simulink model "Communication_rate_control"  (R2025a)
settings: Solver=VariableStepAuto  StartTime=0.0  StopTime=30  RelTol=1e-3
InitFcn:
  | %% Simulation parameters and waypoint trajectory
  | % Initial drone positions.
  | init_0=[0;0;0];
  | d_s=4;
  | init_1=init_0+d_s*[-1;0.1;0];
  | init_2=init_0+d_s*[0.3;-2;0];
  | init_3=init_0+d_s*[0.2;3;0];
  | init_4=init_0+d_s*[4;0.4;0];
  | 
  | Threshold = 1000*ones(45,1);
  | for i=1:9:37
  |     Threshold(i:i+2)=10;
  | end
  | gain_2=1;
  | 
  | % PID controller gains.
  | PID_p=20;
  | PID_i=50;
  | PID_d=0;
  | 
  | % Router queues and background traffic.
  | router_buffer=50;
  | router_bandwith=25;
  | router_init_queue=[2,0,0,0,0];
  | traffic_mean=20;
  | traffic_variance=1;
  | 
  | 
  | % Desired formation offsets.
  | init_f_0=[0;0;0];
  | d_f=1;
  | init_f_1=init_0+d_f*[-1;0;0];
  | init_f_2=init_0+d_f*[0;-1;0];
  | init_f_3=init_0+d_f*[0;1;0];
  | init_f_4=init_0+d_f*[1;0;0];
  | 
  | % Quadrotor mass and inertia.
  | mass = 1.2;
  | Ib   = diag([1.2416 1.2416 2*1.2416]);
  | 
  | % Time grid and waypoint trajectory.
  | Ts        = 0.001;
  | ttot      = 20;
  | tdead     = 10;
  | totalTime = ttot + tdead;
  | Nsamples  = 3000;
  | t_sample  = linspace(0, totalTime, Nsamples);
  | t=t_sample;
  | waypoints = [ ...
  |              0  0 -2 0;
  |              3  4 -5 0;
  |              2  1 -8 0;
  |              0 0 -20 0];
  | 
  | M    = size(waypoints,1);
  | t_wp = linspace(0, ttot, M);
  | 
  | p_d      = zeros(4, Nsamples);
  | dot_p_d  = zeros(4, Nsamples);
  | ddot_p_d = zeros(4, Nsamples);
  | ... (+33 lines)
undefined symbols (not defined in the file): A_diacenza, DiscIntNeverNeededParam, K, L
libraries: dspsigops x10, robotcorelib x5, slpidlib x5, dspstat3 x5, uavutilslib x1
(part 2 of 3)

== system Communication_rate_control/Subsystem1/Subsystem_5 ==
  References : Inport
  Coordinate Transformation Conversion : robotcorelib/Coordinate Transformation Conversion  InputRepresentation=Rotation Matrix  InputEulerSequence=ZYX  ShowTrVecInputPort=on  OutputRepresentation=Quaternion  OutputEulerSequence=ZYX  ShowTrVecOutputPort=on  SimulateUsing=Interpreted execution
  Inner-loop control : Subsystem
  Outer-loop control : MATLAB Function  TreatAsAtomicUnit=on
  Planner : Subsystem
  Quadrotor dynamics : Subsystem
  Scope{,1..5} (6 alike) : Scope
      Scope settings: ActiveDisplayYMinimum=-1.2E-5  ActiveDisplayYMaximum=1.2E-5
      Scope1 settings: ActiveDisplayYMinimum=-1.2E-5  ActiveDisplayYMaximum=1.2E-5
      Scope2 settings: ActiveDisplayYMinimum=-3.9E-5  ActiveDisplayYMaximum=1.1E-5  DataLoggingVariableName=ScopeData2
      Scope3 settings: ActiveDisplayYMinimum=-0.00022  ActiveDisplayYMaximum=0.00011  DataLoggingVariableName=ScopeData3
      Scope4 settings: ActiveDisplayYMinimum=11.66748  ActiveDisplayYMaximum=12.03695  DataLoggingVariableName=ScopeData4
      Scope5 settings: ActiveDisplayYMinimum=-0.02035  ActiveDisplayYMaximum=0.02036  DataLoggingVariableName=ScopeData5
  Terminator : Terminator
  Terminator3 : Terminator
  Unit Delay1 u0=12N : UnitDelay  InitialCondition=12  SampleTime=Ts
  Unit Delay2 : UnitDelay  InitialCondition=[0 0 0]  SampleTime=Ts
  Zero-Order Hold{1..5} (5 alike) : ZeroOrderHold  SampleTime=Ts
  Lin Acc : Outport
  Lin Vel : Outport  Port=2
  Lin Pos : Outport  Port=3
  Rotation : Outport  Port=4
  wires:
  Zero-Order Hold5/1 -> Lin Acc/1
  Quadrotor dynamics/7(lin_acc) -> Zero-Order Hold5/1
  Planner/1(position_des) -> Outer-loop control/4(position_des)
  Quadrotor dynamics/1(Position) -> Zero-Order Hold4/1
  Quadrotor dynamics/3(Rb) -> Zero-Order Hold2/1, Coordinate Transformation Conversion/1
  Quadrotor dynamics/4(dot_Rb) -> Terminator/1
  Planner/4(xb_des) -> Inner-loop control/4(xb_des)
  Inner-loop control/1(tau) -> Unit Delay2/1
  Planner/2(linear_velocity_des) -> Outer-loop control/5(vel_linear_des)
  Quadrotor dynamics/2(Linear_velocity) -> Zero-Order Hold1/1
  Quadrotor dynamics/6(dot_omega_bb) -> Terminator3/1
  Outer-loop control/3(err_p) -> Scope2/1
  Coordinate Transformation Conversion/1 -> Rotation/1
  Quadrotor dynamics/5(omega_bb) -> Zero-Order Hold3/1
  Zero-Order Hold2/1 -> Inner-loop control/2(Rb), Outer-loop control/3(Rb)
  References/1 -> Planner/1(References)
  Planner/3(linear_acceleration_des) -> Outer-loop control/6(acc_linear_des)
  Inner-loop control/3(err_W) -> Scope1/1
  Outer-loop control/2(zb_des) -> Inner-loop control/1(zb_des)
  Inner-loop control/2(err_R) -> Scope/1
  Outer-loop control/1(uT) -> Unit Delay1 u0=12N/1
  Unit Delay2/1 -> Quadrotor dynamics/2(tau_b), Scope5/1
  Zero-Order Hold3/1 -> Inner-loop control/3(omega_bb)
  Unit Delay1 u0=12N/1 -> Scope4/1, Quadrotor dynamics/1(uT)
  Outer-loop control/4(dot_err_p) -> Scope3/1
  Zero-Order Hold1/1 -> Outer-loop control/2(linear_vel), Lin Vel/1
  Zero-Order Hold4/1 -> Outer-loop control/1(position), Lin Pos/1

== system Communication_rate_control/Subsystem13/Planner ==
  Constant : Constant  Value=0
  Mux{1..4} (4 alike) : Mux  Inputs=3
  Trigonometric Function : Trigonometry
  Trigonometric Function1 : Trigonometry  Operator=cos
  ddot_x_d : FromWorkspace  VariableName=[t' ddot_csi_d(1,:)']  SampleTime=Ts
  ddot_y_d : FromWorkspace  VariableName=[t' ddot_csi_d(2,:)']  SampleTime=Ts
  ddot_z_d : FromWorkspace  VariableName=[t' ddot_csi_d(3,:)']  SampleTime=Ts
  dot_x_d1 : FromWorkspace  VariableName=[t' dot_csi_d(1,:)']  SampleTime=Ts
  dot_y_d1 : FromWorkspace  VariableName=[t' dot_csi_d(2,:)']  SampleTime=Ts
  dot_z_d1 : FromWorkspace  VariableName=[t' dot_csi_d(3,:)']  SampleTime=Ts
  psi_d1 : FromWorkspace  VariableName=[t' psi_d']  SampleTime=Ts
  x_d : FromWorkspace  VariableName=[t' csi_d(1,:)']  SampleTime=Ts
  y_d : FromWorkspace  VariableName=[t' csi_d(2,:)']  SampleTime=Ts
  z_d : FromWorkspace  VariableName=[t' csi_d(3,:)']  SampleTime=Ts
  position_des : Outport
  linear_velocity_des : Outport  Port=2
  linear_acceleration_des : Outport  Port=3
  xb_des : Outport  Port=4
  wires:
  y_d/1 -> Mux1/2
  z_d/1 -> Mux1/3
  x_d/1 -> Mux1/1
  ddot_y_d/1 -> Mux2/2
  ddot_z_d/1 -> Mux2/3
  ddot_x_d/1 -> Mux2/1
  Mux2/1 -> linear_acceleration_des/1
  Mux1/1 -> position_des/1
  dot_y_d1/1 -> Mux3/2
  dot_z_d1/1 -> Mux3/3
  dot_x_d1/1 -> Mux3/1
  Mux3/1 -> linear_velocity_des/1
  Mux4/1 -> xb_des/1
  Trigonometric Function/1 -> Mux4/2
  psi_d1/1 -> Trigonometric Function/1, Trigonometric Function1/1
  Trigonometric Function1/1 -> Mux4/1
  Constant/1 -> Mux4/3

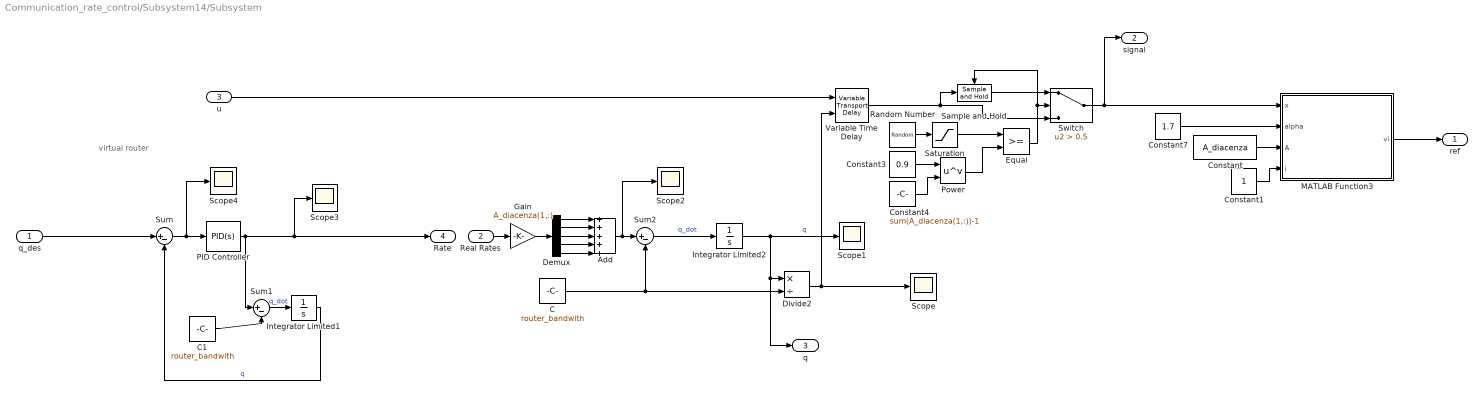
== system Communication_rate_control/Subsystem14/Subsystem ==
  note: virtual router
  q_des : Inport
  " Real Rates" : Inport  Port=2
  u : Inport  Port=3
  Add : Sum  Inputs=+++++
  C : Constant  Value=router_bandwith
  C1 : Constant  Value=router_bandwith
  Constant : Constant  Value=A_diacenza
  Constant1 : Constant
  Constant3 : Constant  Value=0.9
  Constant4 : Constant  Value=sum(A_diacenza(1,:))-1
  Constant7 : Constant  Value=1.7
  Demux : Demux  Outputs=5
  Divide2 : Product  Inputs=*/
  Equal : RelationalOperator  OutDataTypeStr=boolean  RndMeth=Simplest  InputSameDT=off
  Gain : Gain  Gain=A_diacenza(1,:)
  Integrator Limited1 : Integrator  InitialCondition=router_init_queue(1)  LimitOutput=on  UpperSaturationLimit=router_buffer  LowerSaturationLimit=0
  Integrator Limited2 : Integrator  InitialCondition=router_init_queue(1)  LimitOutput=on  UpperSaturationLimit=router_buffer  LowerSaturationLimit=0
  MATLAB Function3 : MATLAB Function  TreatAsAtomicUnit=on
  PID Controller : slpidlib/PID Controller  Controller=PID  Form=Parallel  TimeDomain=Continuous-time  UseExternalTs=off  SampleTime=-1  IntegratorMethod=Forward Euler  FilterMethod=Forward Euler  ControllerParametersSource=internal  P=PID_p  I=PID_i  UseKiTs=off  D=PID_d  UseExternalDerivativeSource=off  N=100  UseFilter=on  TunerSelectOption=Transfer Function Based (PID Tuner App)  InitialConditionSource=internal  InitialConditionForIntegrator=0  InitialConditionForFilter=0  DifferentiatorICPrevScaledInput=0  ExternalReset=none  TrackingMode=off  Kt=1  LimitOutput=off  SatLimitsSource=internal  UpperSaturationLimit=inf  LowerSaturationLimit=-inf  LinearizeAsGain=on  AntiWindupMode=none  Kb=1  LimitIntegrator=off  UpperIntegratorSaturationLimit=inf  LowerIntegratorSaturationLimit=-inf  POutMin=[]  POutMax=[]  IOutMin=[]  IOutMax=[]  DOutMin=[]  DOutMax=[]  NOutMin=[]  NOutMax=[]  SumOutMin=[]  SumOutMax=[]  SaturationOutMin=[]  SaturationOutMax=[]  PParamMin=[]  PParamMax=[]  IParamMin=[]  IParamMax=[]  DParamMin=[]  DParamMax=[]  NParamMin=[]  NParamMax=[]  KbParamMin=[]  KbParamMax=[]  KtParamMin=[]  KtParamMax=[]  KbOutMin=[]  KbOutMax=[]  KtOutMin=[]  KtOutMax=[]  IntegratorOutMin=[]  IntegratorOutMax=[]  FilterOutMin=[]  FilterOutMax=[]  SumI1OutMin=[]  SumI1OutMax=[]  SumI2OutMin=[]  SumI2OutMax=[]  SumI3OutMin=[]  SumI3OutMax=[]  SumI4OutMin=[]  SumI4OutMax=[]  SumDOutMin=[]  SumDOutMax=[]  DifferentiatorOutMin=[]  DifferentiatorOutMax=[]  FilterDiffOutCoefMin=[]  FilterDiffOutCoefMax=[]  ReciprocalOutMin=[]  ReciprocalOutMax=[]  SumDenOutMin=[]  SumDenOutMax=[]  SumNumOutMin=[]  SumNumOutMax=[]  DivideOutMin=[]  DivideOutMax=[]  UdiffTsProdOutMin=[]  UdiffTsProdOutMax=[]  NTsProdOutMin=[]  NTsProdOutMax=[]  UintegralTsProdOutMin=[]  UintegralTsProdOutMax=[]  UngainTsProdOutMin=[]  UngainTsProdOutMax=[]  ClampingZeroOutDataTypeStr=Inherit: Inherit via back propagation  ClampingZeroOutMin=[]  ClampingZeroOutMax=[]  FilterDenConstantOutDataTypeStr=Inherit: Inherit via back propagation  FilterDenConstantOutMin=[]  FilterDenConstantOutMax=[]  PCopyOutDataTypeStr=Inherit: Inherit via back propagation  PCopyOutMin=[]  PCopyOutMax=[]  NCopyOutDataTypeStr=Inherit: Inherit via back propagation  NCopyOutMin=[]  NCopyOutMax=[]  IntegratorContinuousStateAttributes=''  IntegratorStateMustResolveToSignalObject=off  IntegratorRTWStateStorageClass=Auto  FilterContinuousStateAttributes=''  FilterStateMustResolveToSignalObject=off  FilterRTWStateStorageClass=Auto  ParallelPVariant=InternalParameters  IdealPVariant=Disabled  IVariant=InternalParameters  DVariant=InternalParameters  IntegratorVariant=Continuous  SatVariant=Disabled  AWVariant=Passthrough  PCopyVariant=Disabled  TRVariant=Disabled  FdbkBlocksVariant=Forward  IdealPFdbkVariant=Disabled  SatFdbkVariant=Disabled  DerivativeFilterVariant=ContFilter  NVariant=InternalParameters  NCopyVariant=Disabled  FilterICVariant=InternalICsFilter  IntegratorICVariant=InternalICs  ExternalResetVariant=Disabled  TRSumVariant=Passthrough  SumFdbkVariant=Disabled  SumVariant=Sum_PID  TsampFilterVariant=InternalTs  TsampNgainVariant=Passthrough  TsampIntegralVariant=Disabled_SignalSpec  ExternalSaturationOutDataTypeStr=Inherit: Same as second input  DerivativeSourceVariant=ErrorSignal  PreIntVariant=InternalPreInt
  Power : Math  Operator=pow
  Random Number : RandomNumber  Mean=0.5  Variance=0.5  SampleTime=0.1
  Sample and Hold : dspsigops/Sample and Hold  trig=Rising edge  initCond=0  latchinput=off
  Saturation : Saturate  UpperLimit=1  LowerLimit=0
  Scope{,1..4} (5 alike) : Scope
      Scope settings: ActiveDisplayYMinimum=-1  ActiveDisplayYMaximum=1  DataLoggingVariableName=ScopeData7
      Scope1 settings: ActiveDisplayYMinimum=-1  ActiveDisplayYMaximum=1  DataLoggingVariableName=ScopeData8
      Scope2 settings: ActiveDisplayYMinimum=13.95346208966077  ActiveDisplayYMaximum=109.54638870962908  DataLoggingVariableName=ScopeData13
      Scope3 settings: ActiveDisplayYMinimum=18.031914924971169  ActiveDisplayYMaximum=21.223404282118214  DataLoggingVariableName=ScopeData12
      Scope4 settings: ActiveDisplayYMinimum=-3.625  ActiveDisplayYMaximum=2.625  DataLoggingVariableName=ScopeData29
  Sum : Sum  Inputs=|+-
  Sum1 : Sum  Inputs=|+-
  Sum2 : Sum  Inputs=|+-
  Switch : Switch  Criteria=u2 > Threshold  Threshold=0.5  SaturateOnIntegerOverflow=off  InputSameDT=off
  Variable Time Delay : VariableTransportDelay  MaximumDelay=1000  InitialOutput=[init_0;zeros(6,1);init_1;zeros(6,1);init_2;zeros(6,1);init_3;zeros(6,1);init_4;zeros(6,1);]  MaximumPoints=1e4  ZeroDelay=on
  ref : Outport
  "signal " : Outport  Port=2
  q : Outport  Port=3
  " Rate" : Outport  Port=4
  wires:
  Constant7/1 -> MATLAB Function3/2(alpha)
  Constant/1 -> MATLAB Function3/3(A)
  Constant1/1 -> MATLAB Function3/4(i)
  MATLAB Function3/1(vi) -> ref/1
  Integrator Limited2/1 -> q/1, Divide2/1, Scope1/1  "q"
  Switch/1 -> "signal "/1, MATLAB Function3/1(x)
  u/1 -> Variable Time Delay/1
  Sum2/1 -> Integrator Limited2/1  "q_dot"
  Divide2/1 -> Scope/1, Variable Time Delay/2
  C/1 -> Divide2/2, Sum2/2
  Variable Time Delay/1 -> Sample and Hold/1, Switch/3
  PID Controller/1 -> Sum1/1, " Rate"/1, Scope3/1
  Sum/1 -> Scope4/1, PID Controller/1
  q_des/1 -> Sum/1
  Sum1/1 -> Integrator Limited1/1  "q_dot"
  Integrator Limited1/1 -> Sum/2  "q"
  C1/1 -> Sum1/2
  Demux/3 -> Add/3
  Demux/4 -> Add/4
  Demux/2 -> Add/2
  Demux/5 -> Add/5
  Demux/1 -> Add/1
  Add/1 -> Scope2/1, Sum2/1
  " Real Rates"/1 -> Gain/1
  Gain/1 -> Demux/1
  Random Number/1 -> Saturation/1
  Equal/1 -> Sample and Hold/Trigger, Switch/2
  Power/1 -> Equal/2
  Saturation/1 -> Equal/1
  Constant3/1 -> Power/1
  Constant4/1 -> Power/2
  Sample and Hold/1 -> Switch/1

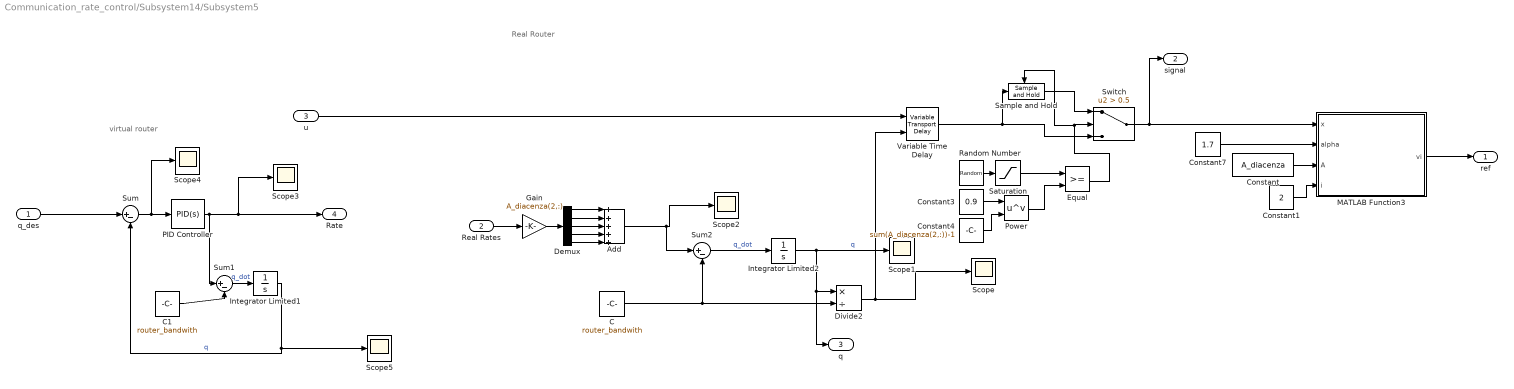
== system Communication_rate_control/Subsystem14/Subsystem5 ==
  note: Real Router
  note: virtual router
  q_des : Inport
  " Real Rates" : Inport  Port=2
  u : Inport  Port=3
  Add : Sum  Inputs=+++++
  C : Constant  Value=router_bandwith
  C1 : Constant  Value=router_bandwith
  Constant : Constant  Value=A_diacenza
  Constant1 : Constant  Value=2
  Constant3 : Constant  Value=0.9
  Constant4 : Constant  Value=sum(A_diacenza(2,:))-1
  Constant7 : Constant  Value=1.7
  Demux : Demux  Outputs=5
  Divide2 : Product  Inputs=*/
  Equal : RelationalOperator  OutDataTypeStr=boolean  RndMeth=Simplest  InputSameDT=off
  Gain : Gain  Gain=A_diacenza(2,:)
  Integrator Limited1 : Integrator  InitialCondition=router_init_queue(1)  LimitOutput=on  UpperSaturationLimit=router_buffer  LowerSaturationLimit=0
  Integrator Limited2 : Integrator  InitialCondition=router_init_queue(2)  LimitOutput=on  UpperSaturationLimit=router_buffer  LowerSaturationLimit=0
  MATLAB Function3 : MATLAB Function  TreatAsAtomicUnit=on
  PID Controller : slpidlib/PID Controller  Controller=PID  Form=Parallel  TimeDomain=Continuous-time  UseExternalTs=off  SampleTime=-1  IntegratorMethod=Forward Euler  FilterMethod=Forward Euler  ControllerParametersSource=internal  P=PID_p  I=PID_i  UseKiTs=off  D=PID_d  UseExternalDerivativeSource=off  N=100  UseFilter=on  TunerSelectOption=Transfer Function Based (PID Tuner App)  InitialConditionSource=internal  InitialConditionForIntegrator=0  InitialConditionForFilter=0  DifferentiatorICPrevScaledInput=0  ExternalReset=none  TrackingMode=off  Kt=1  LimitOutput=off  SatLimitsSource=internal  UpperSaturationLimit=inf  LowerSaturationLimit=-inf  LinearizeAsGain=on  AntiWindupMode=none  Kb=1  LimitIntegrator=off  UpperIntegratorSaturationLimit=inf  LowerIntegratorSaturationLimit=-inf  POutMin=[]  POutMax=[]  IOutMin=[]  IOutMax=[]  DOutMin=[]  DOutMax=[]  NOutMin=[]  NOutMax=[]  SumOutMin=[]  SumOutMax=[]  SaturationOutMin=[]  SaturationOutMax=[]  PParamMin=[]  PParamMax=[]  IParamMin=[]  IParamMax=[]  DParamMin=[]  DParamMax=[]  NParamMin=[]  NParamMax=[]  KbParamMin=[]  KbParamMax=[]  KtParamMin=[]  KtParamMax=[]  KbOutMin=[]  KbOutMax=[]  KtOutMin=[]  KtOutMax=[]  IntegratorOutMin=[]  IntegratorOutMax=[]  FilterOutMin=[]  FilterOutMax=[]  SumI1OutMin=[]  SumI1OutMax=[]  SumI2OutMin=[]  SumI2OutMax=[]  SumI3OutMin=[]  SumI3OutMax=[]  SumI4OutMin=[]  SumI4OutMax=[]  SumDOutMin=[]  SumDOutMax=[]  DifferentiatorOutMin=[]  DifferentiatorOutMax=[]  FilterDiffOutCoefMin=[]  FilterDiffOutCoefMax=[]  ReciprocalOutMin=[]  ReciprocalOutMax=[]  SumDenOutMin=[]  SumDenOutMax=[]  SumNumOutMin=[]  SumNumOutMax=[]  DivideOutMin=[]  DivideOutMax=[]  UdiffTsProdOutMin=[]  UdiffTsProdOutMax=[]  NTsProdOutMin=[]  NTsProdOutMax=[]  UintegralTsProdOutMin=[]  UintegralTsProdOutMax=[]  UngainTsProdOutMin=[]  UngainTsProdOutMax=[]  ClampingZeroOutDataTypeStr=Inherit: Inherit via back propagation  ClampingZeroOutMin=[]  ClampingZeroOutMax=[]  FilterDenConstantOutDataTypeStr=Inherit: Inherit via back propagation  FilterDenConstantOutMin=[]  FilterDenConstantOutMax=[]  PCopyOutDataTypeStr=Inherit: Inherit via back propagation  PCopyOutMin=[]  PCopyOutMax=[]  NCopyOutDataTypeStr=Inherit: Inherit via back propagation  NCopyOutMin=[]  NCopyOutMax=[]  IntegratorContinuousStateAttributes=''  IntegratorStateMustResolveToSignalObject=off  IntegratorRTWStateStorageClass=Auto  FilterContinuousStateAttributes=''  FilterStateMustResolveToSignalObject=off  FilterRTWStateStorageClass=Auto  ParallelPVariant=InternalParameters  IdealPVariant=Disabled  IVariant=InternalParameters  DVariant=InternalParameters  IntegratorVariant=Continuous  SatVariant=Disabled  AWVariant=Passthrough  PCopyVariant=Disabled  TRVariant=Disabled  FdbkBlocksVariant=Forward  IdealPFdbkVariant=Disabled  SatFdbkVariant=Disabled  DerivativeFilterVariant=ContFilter  NVariant=InternalParameters  NCopyVariant=Disabled  FilterICVariant=InternalICsFilter  IntegratorICVariant=InternalICs  ExternalResetVariant=Disabled  TRSumVariant=Passthrough  SumFdbkVariant=Disabled  SumVariant=Sum_PID  TsampFilterVariant=InternalTs  TsampNgainVariant=Passthrough  TsampIntegralVariant=Disabled_SignalSpec  ExternalSaturationOutDataTypeStr=Inherit: Same as second input  DerivativeSourceVariant=ErrorSignal  PreIntVariant=InternalPreInt
  Power : Math  Operator=pow
  Random Number : RandomNumber  Mean=0.5  Variance=0.5  SampleTime=0.1
  Sample and Hold : dspsigops/Sample and Hold  trig=Rising edge  initCond=0  latchinput=off
  Saturation : Saturate  UpperLimit=1  LowerLimit=0
  Scope{,1..5} (6 alike) : Scope
      Scope settings: DataLoggingVariableName=ScopeData7
      Scope1 settings: ActiveDisplayYMinimum=-1  ActiveDisplayYMaximum=1  DataLoggingVariableName=ScopeData8
      Scope2 settings: ActiveDisplayYMinimum=-4.9997275794883738  ActiveDisplayYMaximum=44.997548215395369  DataLoggingVariableName=ScopeData13
      Scope3 settings: ActiveDisplayYMinimum=-48.354575152001019  ActiveDisplayYMaximum=35.191176368009138  DataLoggingVariableName=ScopeData14
      Scope4 settings: ActiveDisplayYMinimum=-3.625  ActiveDisplayYMaximum=2.625  DataLoggingVariableName=ScopeData15
      Scope5 settings: ActiveDisplayYMinimum=-0.24999999999999994  ActiveDisplayYMaximum=2.25  DataLoggingVariableName=ScopeData25
  Sum : Sum  Inputs=|+-
  Sum1 : Sum  Inputs=|+-
  Sum2 : Sum  Inputs=|+-
  Switch : Switch  Criteria=u2 > Threshold  Threshold=0.5  SaturateOnIntegerOverflow=off  InputSameDT=off
  Variable Time Delay : VariableTransportDelay  MaximumDelay=1000  InitialOutput=[init_0;zeros(6,1);init_1;zeros(6,1);init_2;zeros(6,1);init_3;zeros(6,1);init_4;zeros(6,1);]  MaximumPoints=1e4  ZeroDelay=on
  ref : Outport
  "signal " : Outport  Port=2
  q : Outport  Port=3
  " Rate" : Outport  Port=4
  wires:
  Sample and Hold/1 -> Switch/1
  Variable Time Delay/1 -> Sample and Hold/1, Switch/3
  C/1 -> Sum2/2, Divide2/2
  Divide2/1 -> Variable Time Delay/2, Scope/1
  Sum2/1 -> Integrator Limited2/1  "q_dot"
  u/1 -> Variable Time Delay/1
  Switch/1 -> MATLAB Function3/1(x), "signal "/1
  Integrator Limited2/1 -> Divide2/1, q/1, Scope1/1  "q"
  MATLAB Function3/1(vi) -> ref/1
  Constant1/1 -> MATLAB Function3/4(i)
  Constant/1 -> MATLAB Function3/3(A)
  Constant7/1 -> MATLAB Function3/2(alpha)
  PID Controller/1 -> " Rate"/1, Scope3/1, Sum1/1
  q_des/1 -> Sum/1
  Sum1/1 -> Integrator Limited1/1  "q_dot"
  Sum/1 -> Scope4/1, PID Controller/1
  C1/1 -> Sum1/2
  Integrator Limited1/1 -> Scope5/1, Sum/2  "q"
  Demux/3 -> Add/3
  Demux/2 -> Add/2
  " Real Rates"/1 -> Gain/1
  Demux/4 -> Add/4
  Demux/5 -> Add/5
  Demux/1 -> Add/1
  Gain/1 -> Demux/1
  Add/1 -> Sum2/1, Scope2/1
  Power/1 -> Equal/2
  Saturation/1 -> Equal/1
  Constant3/1 -> Power/1
  Random Number/1 -> Saturation/1
  Constant4/1 -> Power/2
  Equal/1 -> Sample and Hold/Trigger, Switch/2

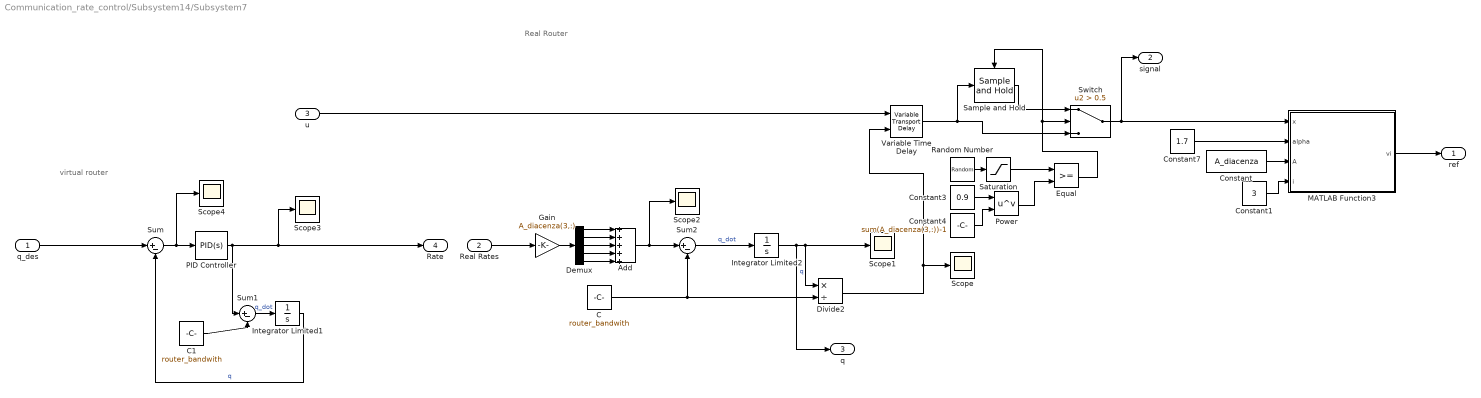
== system Communication_rate_control/Subsystem14/Subsystem7 ==
  note: Real Router
  note: virtual router
  q_des : Inport
  " Real Rates" : Inport  Port=2
  u : Inport  Port=3
  Add : Sum  Inputs=+++++
  C : Constant  Value=router_bandwith
  C1 : Constant  Value=router_bandwith
  Constant : Constant  Value=A_diacenza
  Constant1 : Constant  Value=3
  Constant3 : Constant  Value=0.9
  Constant4 : Constant  Value=sum(A_diacenza(3,:))-1
  Constant7 : Constant  Value=1.7
  Demux : Demux  Outputs=5
  Divide2 : Product  Inputs=*/
  Equal : RelationalOperator  OutDataTypeStr=boolean  RndMeth=Simplest  InputSameDT=off
  Gain : Gain  Gain=A_diacenza(3,:)
  Integrator Limited1 : Integrator  InitialCondition=router_init_queue(1)  LimitOutput=on  UpperSaturationLimit=router_buffer  LowerSaturationLimit=0
  Integrator Limited2 : Integrator  InitialCondition=router_init_queue(3)  LimitOutput=on  UpperSaturationLimit=router_buffer  LowerSaturationLimit=0
  MATLAB Function3 : MATLAB Function  TreatAsAtomicUnit=on
  PID Controller : slpidlib/PID Controller  Controller=PID  Form=Parallel  TimeDomain=Continuous-time  UseExternalTs=off  SampleTime=-1  IntegratorMethod=Forward Euler  FilterMethod=Forward Euler  ControllerParametersSource=internal  P=PID_p  I=PID_i  UseKiTs=off  D=PID_d  UseExternalDerivativeSource=off  N=100  UseFilter=on  TunerSelectOption=Transfer Function Based (PID Tuner App)  InitialConditionSource=internal  InitialConditionForIntegrator=0  InitialConditionForFilter=0  DifferentiatorICPrevScaledInput=0  ExternalReset=none  TrackingMode=off  Kt=1  LimitOutput=off  SatLimitsSource=internal  UpperSaturationLimit=inf  LowerSaturationLimit=-inf  LinearizeAsGain=on  AntiWindupMode=none  Kb=1  LimitIntegrator=off  UpperIntegratorSaturationLimit=inf  LowerIntegratorSaturationLimit=-inf  POutMin=[]  POutMax=[]  IOutMin=[]  IOutMax=[]  DOutMin=[]  DOutMax=[]  NOutMin=[]  NOutMax=[]  SumOutMin=[]  SumOutMax=[]  SaturationOutMin=[]  SaturationOutMax=[]  PParamMin=[]  PParamMax=[]  IParamMin=[]  IParamMax=[]  DParamMin=[]  DParamMax=[]  NParamMin=[]  NParamMax=[]  KbParamMin=[]  KbParamMax=[]  KtParamMin=[]  KtParamMax=[]  KbOutMin=[]  KbOutMax=[]  KtOutMin=[]  KtOutMax=[]  IntegratorOutMin=[]  IntegratorOutMax=[]  FilterOutMin=[]  FilterOutMax=[]  SumI1OutMin=[]  SumI1OutMax=[]  SumI2OutMin=[]  SumI2OutMax=[]  SumI3OutMin=[]  SumI3OutMax=[]  SumI4OutMin=[]  SumI4OutMax=[]  SumDOutMin=[]  SumDOutMax=[]  DifferentiatorOutMin=[]  DifferentiatorOutMax=[]  FilterDiffOutCoefMin=[]  FilterDiffOutCoefMax=[]  ReciprocalOutMin=[]  ReciprocalOutMax=[]  SumDenOutMin=[]  SumDenOutMax=[]  SumNumOutMin=[]  SumNumOutMax=[]  DivideOutMin=[]  DivideOutMax=[]  UdiffTsProdOutMin=[]  UdiffTsProdOutMax=[]  NTsProdOutMin=[]  NTsProdOutMax=[]  UintegralTsProdOutMin=[]  UintegralTsProdOutMax=[]  UngainTsProdOutMin=[]  UngainTsProdOutMax=[]  ClampingZeroOutDataTypeStr=Inherit: Inherit via back propagation  ClampingZeroOutMin=[]  ClampingZeroOutMax=[]  FilterDenConstantOutDataTypeStr=Inherit: Inherit via back propagation  FilterDenConstantOutMin=[]  FilterDenConstantOutMax=[]  PCopyOutDataTypeStr=Inherit: Inherit via back propagation  PCopyOutMin=[]  PCopyOutMax=[]  NCopyOutDataTypeStr=Inherit: Inherit via back propagation  NCopyOutMin=[]  NCopyOutMax=[]  IntegratorContinuousStateAttributes=''  IntegratorStateMustResolveToSignalObject=off  IntegratorRTWStateStorageClass=Auto  FilterContinuousStateAttributes=''  FilterStateMustResolveToSignalObject=off  FilterRTWStateStorageClass=Auto  ParallelPVariant=InternalParameters  IdealPVariant=Disabled  IVariant=InternalParameters  DVariant=InternalParameters  IntegratorVariant=Continuous  SatVariant=Disabled  AWVariant=Passthrough  PCopyVariant=Disabled  TRVariant=Disabled  FdbkBlocksVariant=Forward  IdealPFdbkVariant=Disabled  SatFdbkVariant=Disabled  DerivativeFilterVariant=ContFilter  NVariant=InternalParameters  NCopyVariant=Disabled  FilterICVariant=InternalICsFilter  IntegratorICVariant=InternalICs  ExternalResetVariant=Disabled  TRSumVariant=Passthrough  SumFdbkVariant=Disabled  SumVariant=Sum_PID  TsampFilterVariant=InternalTs  TsampNgainVariant=Passthrough  TsampIntegralVariant=Disabled_SignalSpec  ExternalSaturationOutDataTypeStr=Inherit: Same as second input  DerivativeSourceVariant=ErrorSignal  PreIntVariant=InternalPreInt
  Power : Math  Operator=pow
  Random Number : RandomNumber  Mean=0.5  Variance=0.5  SampleTime=0.1
  Sample and Hold : dspsigops/Sample and Hold  trig=Rising edge  initCond=0  latchinput=off
  Saturation : Saturate  UpperLimit=1  LowerLimit=0
  Scope{,1..4} (5 alike) : Scope
      Scope settings: ActiveDisplayYMinimum=-1  ActiveDisplayYMaximum=1  DataLoggingVariableName=ScopeData7
      Scope1 settings: ActiveDisplayYMinimum=1.4313918245472816  ActiveDisplayYMaximum=3.3975685911844873  DataLoggingVariableName=ScopeData8
      Scope2 settings: ActiveDisplayYMinimum=-5.0715881779365786  ActiveDisplayYMaximum=37.614274886734989  DataLoggingVariableName=ScopeData23
      Scope3 settings: ActiveDisplayYMinimum=18.031914924971169  ActiveDisplayYMaximum=21.223404282118214  DataLoggingVariableName=ScopeData18
      Scope4 settings: ActiveDisplayYMinimum=-3.625  ActiveDisplayYMaximum=2.625  DataLoggingVariableName=ScopeData19
  Sum : Sum  Inputs=|+-
  Sum1 : Sum  Inputs=|+-
  Sum2 : Sum  Inputs=|+-
  Switch : Switch  Criteria=u2 > Threshold  Threshold=0.5  SaturateOnIntegerOverflow=off  InputSameDT=off
  Variable Time Delay : VariableTransportDelay  MaximumDelay=1000  InitialOutput=[init_0;zeros(6,1);init_1;zeros(6,1);init_2;zeros(6,1);init_3;zeros(6,1);init_4;zeros(6,1);]  MaximumPoints=1e4  ZeroDelay=on
  ref : Outport
  "signal " : Outport  Port=2
  q : Outport  Port=3
  " Rate" : Outport  Port=4
  wires:
  Constant7/1 -> MATLAB Function3/2(alpha)
  Constant/1 -> MATLAB Function3/3(A)
  Constant1/1 -> MATLAB Function3/4(i)
  MATLAB Function3/1(vi) -> ref/1
  Integrator Limited2/1 -> q/1, Scope1/1, Divide2/1  "q"
  Switch/1 -> "signal "/1, MATLAB Function3/1(x)
  u/1 -> Variable Time Delay/1
  Sum2/1 -> Integrator Limited2/1  "q_dot"
  Divide2/1 -> Scope/1, Variable Time Delay/2
  C/1 -> Divide2/2, Sum2/2
  Variable Time Delay/1 -> Sample and Hold/1, Switch/3
  Sample and Hold/1 -> Switch/1
  Integrator Limited1/1 -> Sum/2  "q"
  PID Controller/1 -> Sum1/1, " Rate"/1, Scope3/1
  Sum1/1 -> Integrator Limited1/1  "q_dot"
  C1/1 -> Sum1/2
  Sum/1 -> Scope4/1, PID Controller/1
  q_des/1 -> Sum/1
  Demux/3 -> Add/3
  Demux/2 -> Add/2
  " Real Rates"/1 -> Gain/1
  Demux/4 -> Add/4
  Demux/5 -> Add/5
  Demux/1 -> Add/1
  Gain/1 -> Demux/1
  Add/1 -> Scope2/1, Sum2/1
  Power/1 -> Equal/2
  Saturation/1 -> Equal/1
  Constant3/1 -> Power/1
  Random Number/1 -> Saturation/1
  Constant4/1 -> Power/2
  Equal/1 -> Switch/2, Sample and Hold/Trigger

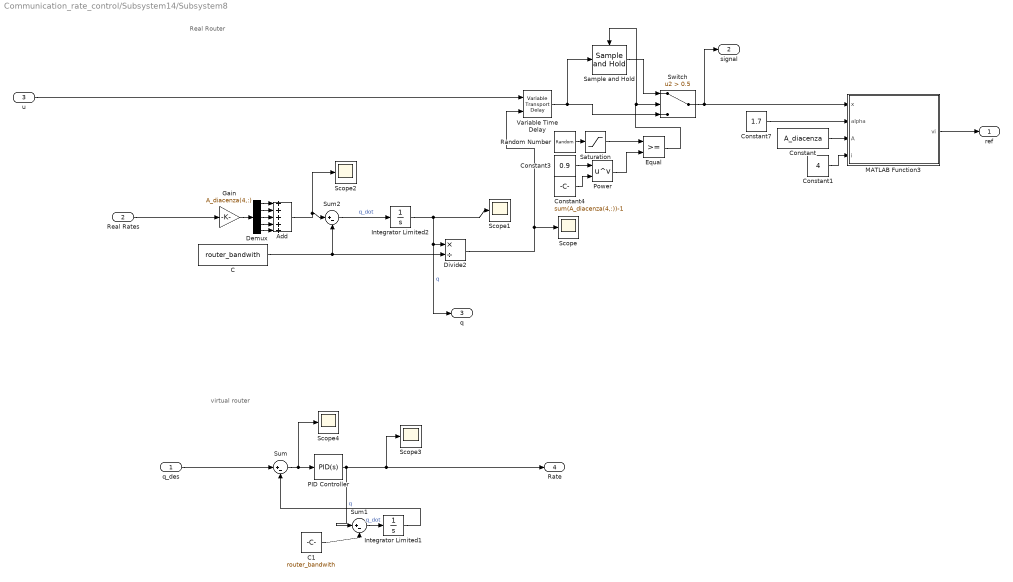
== system Communication_rate_control/Subsystem14/Subsystem8 ==
  note: Real Router
  note: virtual router
  q_des : Inport
  " Real Rates" : Inport  Port=2
  u : Inport  Port=3
  Add : Sum  Inputs=+++++
  C : Constant  Value=router_bandwith
  C1 : Constant  Value=router_bandwith
  Constant : Constant  Value=A_diacenza
  Constant1 : Constant  Value=4
  Constant3 : Constant  Value=0.9
  Constant4 : Constant  Value=sum(A_diacenza(4,:))-1
  Constant7 : Constant  Value=1.7
  Demux : Demux  Outputs=5
  Divide2 : Product  Inputs=*/
  Equal : RelationalOperator  OutDataTypeStr=boolean  RndMeth=Simplest  InputSameDT=off
  Gain : Gain  Gain=A_diacenza(4,:)
  Integrator Limited1 : Integrator  InitialCondition=router_init_queue(1)  LimitOutput=on  UpperSaturationLimit=router_buffer  LowerSaturationLimit=0
  Integrator Limited2 : Integrator  InitialCondition=router_init_queue(4)  LimitOutput=on  UpperSaturationLimit=router_buffer  LowerSaturationLimit=0
  MATLAB Function3 : MATLAB Function  TreatAsAtomicUnit=on
  PID Controller : slpidlib/PID Controller  Controller=PID  Form=Parallel  TimeDomain=Continuous-time  UseExternalTs=off  SampleTime=-1  IntegratorMethod=Forward Euler  FilterMethod=Forward Euler  ControllerParametersSource=internal  P=PID_p  I=PID_i  UseKiTs=off  D=PID_d  UseExternalDerivativeSource=off  N=100  UseFilter=on  TunerSelectOption=Transfer Function Based (PID Tuner App)  InitialConditionSource=internal  InitialConditionForIntegrator=0  InitialConditionForFilter=0  DifferentiatorICPrevScaledInput=0  ExternalReset=none  TrackingMode=off  Kt=1  LimitOutput=off  SatLimitsSource=internal  UpperSaturationLimit=inf  LowerSaturationLimit=-inf  LinearizeAsGain=on  AntiWindupMode=none  Kb=1  LimitIntegrator=off  UpperIntegratorSaturationLimit=inf  LowerIntegratorSaturationLimit=-inf  POutMin=[]  POutMax=[]  IOutMin=[]  IOutMax=[]  DOutMin=[]  DOutMax=[]  NOutMin=[]  NOutMax=[]  SumOutMin=[]  SumOutMax=[]  SaturationOutMin=[]  SaturationOutMax=[]  PParamMin=[]  PParamMax=[]  IParamMin=[]  IParamMax=[]  DParamMin=[]  DParamMax=[]  NParamMin=[]  NParamMax=[]  KbParamMin=[]  KbParamMax=[]  KtParamMin=[]  KtParamMax=[]  KbOutMin=[]  KbOutMax=[]  KtOutMin=[]  KtOutMax=[]  IntegratorOutMin=[]  IntegratorOutMax=[]  FilterOutMin=[]  FilterOutMax=[]  SumI1OutMin=[]  SumI1OutMax=[]  SumI2OutMin=[]  SumI2OutMax=[]  SumI3OutMin=[]  SumI3OutMax=[]  SumI4OutMin=[]  SumI4OutMax=[]  SumDOutMin=[]  SumDOutMax=[]  DifferentiatorOutMin=[]  DifferentiatorOutMax=[]  FilterDiffOutCoefMin=[]  FilterDiffOutCoefMax=[]  ReciprocalOutMin=[]  ReciprocalOutMax=[]  SumDenOutMin=[]  SumDenOutMax=[]  SumNumOutMin=[]  SumNumOutMax=[]  DivideOutMin=[]  DivideOutMax=[]  UdiffTsProdOutMin=[]  UdiffTsProdOutMax=[]  NTsProdOutMin=[]  NTsProdOutMax=[]  UintegralTsProdOutMin=[]  UintegralTsProdOutMax=[]  UngainTsProdOutMin=[]  UngainTsProdOutMax=[]  ClampingZeroOutDataTypeStr=Inherit: Inherit via back propagation  ClampingZeroOutMin=[]  ClampingZeroOutMax=[]  FilterDenConstantOutDataTypeStr=Inherit: Inherit via back propagation  FilterDenConstantOutMin=[]  FilterDenConstantOutMax=[]  PCopyOutDataTypeStr=Inherit: Inherit via back propagation  PCopyOutMin=[]  PCopyOutMax=[]  NCopyOutDataTypeStr=Inherit: Inherit via back propagation  NCopyOutMin=[]  NCopyOutMax=[]  IntegratorContinuousStateAttributes=''  IntegratorStateMustResolveToSignalObject=off  IntegratorRTWStateStorageClass=Auto  FilterContinuousStateAttributes=''  FilterStateMustResolveToSignalObject=off  FilterRTWStateStorageClass=Auto  ParallelPVariant=InternalParameters  IdealPVariant=Disabled  IVariant=InternalParameters  DVariant=InternalParameters  IntegratorVariant=Continuous  SatVariant=Disabled  AWVariant=Passthrough  PCopyVariant=Disabled  TRVariant=Disabled  FdbkBlocksVariant=Forward  IdealPFdbkVariant=Disabled  SatFdbkVariant=Disabled  DerivativeFilterVariant=ContFilter  NVariant=InternalParameters  NCopyVariant=Disabled  FilterICVariant=InternalICsFilter  IntegratorICVariant=InternalICs  ExternalResetVariant=Disabled  TRSumVariant=Passthrough  SumFdbkVariant=Disabled  SumVariant=Sum_PID  TsampFilterVariant=InternalTs  TsampNgainVariant=Passthrough  TsampIntegralVariant=Disabled_SignalSpec  ExternalSaturationOutDataTypeStr=Inherit: Same as second input  DerivativeSourceVariant=ErrorSignal  PreIntVariant=InternalPreInt
  Power : Math  Operator=pow
  Random Number : RandomNumber  Mean=0.5  Variance=0.5  SampleTime=0.1
  Sample and Hold : dspsigops/Sample and Hold  trig=Rising edge  initCond=0  latchinput=off
  Saturation : Saturate  UpperLimit=1  LowerLimit=0
  Scope{,1..4} (5 alike) : Scope
      Scope settings: DataLoggingVariableName=ScopeData7
      Scope1 settings: ActiveDisplayYMinimum=-1  ActiveDisplayYMaximum=1  DataLoggingVariableName=ScopeData8
      Scope2 settings: ActiveDisplayYMinimum=-16.4776588849588  ActiveDisplayYMaximum=28.850052227950371  DataLoggingVariableName=ScopeData13
      Scope3 settings: ActiveDisplayYMinimum=18.031914924971169  ActiveDisplayYMaximum=21.223404282118214  DataLoggingVariableName=ScopeData16
      Scope4 settings: ActiveDisplayYMinimum=-3.625  ActiveDisplayYMaximum=2.625  DataLoggingVariableName=ScopeData17
  Sum : Sum  Inputs=|+-
  Sum1 : Sum  Inputs=|+-
  Sum2 : Sum  Inputs=|+-
  Switch : Switch  Criteria=u2 > Threshold  Threshold=0.5  SaturateOnIntegerOverflow=off  InputSameDT=off
  Variable Time Delay : VariableTransportDelay  MaximumDelay=1000  InitialOutput=[init_0;zeros(6,1);init_1;zeros(6,1);init_2;zeros(6,1);init_3;zeros(6,1);init_4;zeros(6,1);]  MaximumPoints=1e4  ZeroDelay=on
  ref : Outport
  "signal " : Outport  Port=2
  q : Outport  Port=3
  " Rate" : Outport  Port=4
  wires:
  Sample and Hold/1 -> Switch/1
  Variable Time Delay/1 -> Sample and Hold/1, Switch/3
  C/1 -> Sum2/2, Divide2/2
  Divide2/1 -> Variable Time Delay/2, Scope/1
  Sum2/1 -> Integrator Limited2/1  "q_dot"
  u/1 -> Variable Time Delay/1
  Switch/1 -> MATLAB Function3/1(x), "signal "/1
  Integrator Limited2/1 -> Scope1/1, q/1, Divide2/1  "q"
  MATLAB Function3/1(vi) -> ref/1
  Constant1/1 -> MATLAB Function3/4(i)
  Constant/1 -> MATLAB Function3/3(A)
  Constant7/1 -> MATLAB Function3/2(alpha)
  Add/1 -> Scope2/1, Sum2/1
  Integrator Limited1/1 -> Sum/2  "q"
  PID Controller/1 -> Sum1/1, " Rate"/1, Scope3/1
  Sum1/1 -> Integrator Limited1/1  "q_dot"
  C1/1 -> Sum1/2
  Sum/1 -> Scope4/1, PID Controller/1
  q_des/1 -> Sum/1
  Demux/3 -> Add/3
  Demux/2 -> Add/2
  " Real Rates"/1 -> Gain/1
  Demux/4 -> Add/4
  Demux/5 -> Add/5
  Demux/1 -> Add/1
  Gain/1 -> Demux/1
  Power/1 -> Equal/2
  Saturation/1 -> Equal/1
  Constant3/1 -> Power/1
  Random Number/1 -> Saturation/1
  Constant4/1 -> Power/2
  Equal/1 -> Sample and Hold/Trigger, Switch/2

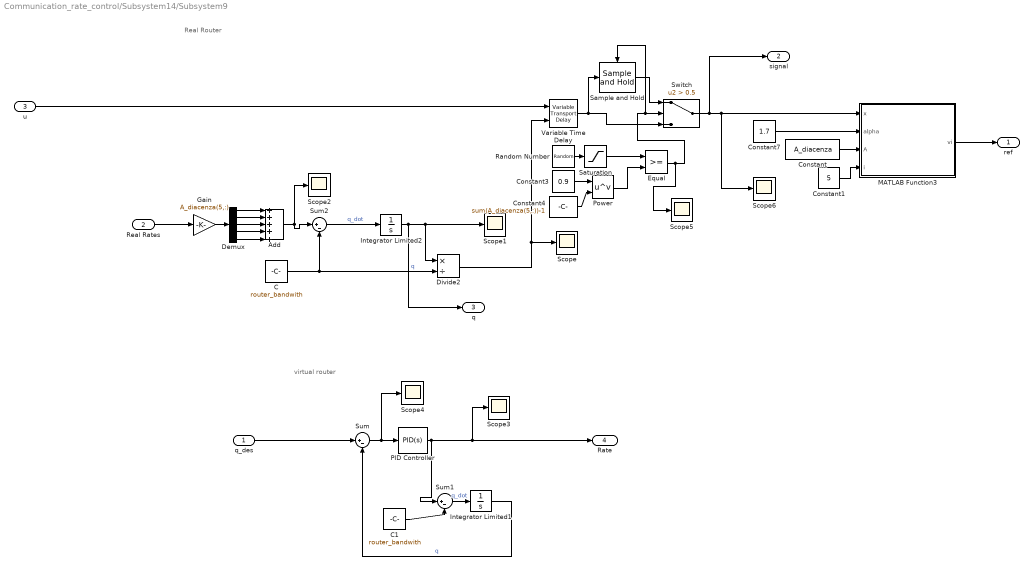
== system Communication_rate_control/Subsystem14/Subsystem9 ==
  note: Real Router
  note: virtual router
  q_des : Inport
  " Real Rates" : Inport  Port=2
  u : Inport  Port=3
  Add : Sum  Inputs=+++++
  C : Constant  Value=router_bandwith
  C1 : Constant  Value=router_bandwith
  Constant : Constant  Value=A_diacenza
  Constant1 : Constant  Value=5
  Constant3 : Constant  Value=0.9
  Constant4 : Constant  Value=sum(A_diacenza(5,:))-1
  Constant7 : Constant  Value=1.7
  Demux : Demux  Outputs=5
  Divide2 : Product  Inputs=*/
  Equal : RelationalOperator  OutDataTypeStr=boolean  RndMeth=Simplest  InputSameDT=off
  Gain : Gain  Gain=A_diacenza(5,:)
  Integrator Limited1 : Integrator  InitialCondition=router_init_queue(1)  LimitOutput=on  UpperSaturationLimit=router_buffer  LowerSaturationLimit=0
  Integrator Limited2 : Integrator  InitialCondition=router_init_queue(5)  LimitOutput=on  UpperSaturationLimit=router_buffer  LowerSaturationLimit=0
  MATLAB Function3 : MATLAB Function  TreatAsAtomicUnit=on
  PID Controller : slpidlib/PID Controller  Controller=PID  Form=Parallel  TimeDomain=Continuous-time  UseExternalTs=off  SampleTime=-1  IntegratorMethod=Forward Euler  FilterMethod=Forward Euler  ControllerParametersSource=internal  P=PID_p  I=PID_i  UseKiTs=off  D=PID_d  UseExternalDerivativeSource=off  N=100  UseFilter=on  TunerSelectOption=Transfer Function Based (PID Tuner App)  InitialConditionSource=internal  InitialConditionForIntegrator=0  InitialConditionForFilter=0  DifferentiatorICPrevScaledInput=0  ExternalReset=none  TrackingMode=off  Kt=1  LimitOutput=off  SatLimitsSource=internal  UpperSaturationLimit=inf  LowerSaturationLimit=-inf  LinearizeAsGain=on  AntiWindupMode=none  Kb=1  LimitIntegrator=off  UpperIntegratorSaturationLimit=inf  LowerIntegratorSaturationLimit=-inf  POutMin=[]  POutMax=[]  IOutMin=[]  IOutMax=[]  DOutMin=[]  DOutMax=[]  NOutMin=[]  NOutMax=[]  SumOutMin=[]  SumOutMax=[]  SaturationOutMin=[]  SaturationOutMax=[]  PParamMin=[]  PParamMax=[]  IParamMin=[]  IParamMax=[]  DParamMin=[]  DParamMax=[]  NParamMin=[]  NParamMax=[]  KbParamMin=[]  KbParamMax=[]  KtParamMin=[]  KtParamMax=[]  KbOutMin=[]  KbOutMax=[]  KtOutMin=[]  KtOutMax=[]  IntegratorOutMin=[]  IntegratorOutMax=[]  FilterOutMin=[]  FilterOutMax=[]  SumI1OutMin=[]  SumI1OutMax=[]  SumI2OutMin=[]  SumI2OutMax=[]  SumI3OutMin=[]  SumI3OutMax=[]  SumI4OutMin=[]  SumI4OutMax=[]  SumDOutMin=[]  SumDOutMax=[]  DifferentiatorOutMin=[]  DifferentiatorOutMax=[]  FilterDiffOutCoefMin=[]  FilterDiffOutCoefMax=[]  ReciprocalOutMin=[]  ReciprocalOutMax=[]  SumDenOutMin=[]  SumDenOutMax=[]  SumNumOutMin=[]  SumNumOutMax=[]  DivideOutMin=[]  DivideOutMax=[]  UdiffTsProdOutMin=[]  UdiffTsProdOutMax=[]  NTsProdOutMin=[]  NTsProdOutMax=[]  UintegralTsProdOutMin=[]  UintegralTsProdOutMax=[]  UngainTsProdOutMin=[]  UngainTsProdOutMax=[]  ClampingZeroOutDataTypeStr=Inherit: Inherit via back propagation  ClampingZeroOutMin=[]  ClampingZeroOutMax=[]  FilterDenConstantOutDataTypeStr=Inherit: Inherit via back propagation  FilterDenConstantOutMin=[]  FilterDenConstantOutMax=[]  PCopyOutDataTypeStr=Inherit: Inherit via back propagation  PCopyOutMin=[]  PCopyOutMax=[]  NCopyOutDataTypeStr=Inherit: Inherit via back propagation  NCopyOutMin=[]  NCopyOutMax=[]  IntegratorContinuousStateAttributes=''  IntegratorStateMustResolveToSignalObject=off  IntegratorRTWStateStorageClass=Auto  FilterContinuousStateAttributes=''  FilterStateMustResolveToSignalObject=off  FilterRTWStateStorageClass=Auto  ParallelPVariant=InternalParameters  IdealPVariant=Disabled  IVariant=InternalParameters  DVariant=InternalParameters  IntegratorVariant=Continuous  SatVariant=Disabled  AWVariant=Passthrough  PCopyVariant=Disabled  TRVariant=Disabled  FdbkBlocksVariant=Forward  IdealPFdbkVariant=Disabled  SatFdbkVariant=Disabled  DerivativeFilterVariant=ContFilter  NVariant=InternalParameters  NCopyVariant=Disabled  FilterICVariant=InternalICsFilter  IntegratorICVariant=InternalICs  ExternalResetVariant=Disabled  TRSumVariant=Passthrough  SumFdbkVariant=Disabled  SumVariant=Sum_PID  TsampFilterVariant=InternalTs  TsampNgainVariant=Passthrough  TsampIntegralVariant=Disabled_SignalSpec  ExternalSaturationOutDataTypeStr=Inherit: Same as second input  DerivativeSourceVariant=ErrorSignal  PreIntVariant=InternalPreInt
  Power : Math  Operator=pow
  Random Number : RandomNumber  Mean=0.5  Variance=0.5  SampleTime=0.1
  Sample and Hold : dspsigops/Sample and Hold  trig=Rising edge  initCond=0  latchinput=off
  Saturation : Saturate  UpperLimit=1  LowerLimit=0
  Scope{,1..6} (7 alike) : Scope
      Scope settings: ActiveDisplayYMinimum=0.0019171133278549479  ActiveDisplayYMaximum=0.066506482659169808  DataLoggingVariableName=ScopeData7
      Scope1 settings: ActiveDisplayYMinimum=-1  ActiveDisplayYMaximum=1  DataLoggingVariableName=ScopeData8
      Scope2 settings: ActiveDisplayYMinimum=-4.9997275794883738  ActiveDisplayYMaximum=44.997548215395369  DataLoggingVariableName=ScopeData13
      Scope3 settings: ActiveDisplayYMinimum=-48.354575152001026  ActiveDisplayYMaximum=35.191176368009216  DataLoggingVariableName=ScopeData20
      Scope4 settings: ActiveDisplayYMinimum=-3.625  ActiveDisplayYMaximum=2.625  DataLoggingVariableName=ScopeData21
      Scope5 settings: ActiveDisplayYMinimum=-1  ActiveDisplayYMaximum=1  DataLoggingVariableName=ScopeData6
      Scope6 settings: ActiveDisplayYMinimum=-1  ActiveDisplayYMaximum=1  DataLoggingVariableName=ScopeData31
  Sum : Sum  Inputs=|+-
  Sum1 : Sum  Inputs=|+-
  Sum2 : Sum  Inputs=|+-
  Switch : Switch  Criteria=u2 > Threshold  Threshold=0.5  SaturateOnIntegerOverflow=off  InputSameDT=off
  Variable Time Delay : VariableTransportDelay  MaximumDelay=1000  InitialOutput=[init_0;zeros(6,1);init_1;zeros(6,1);init_2;zeros(6,1);init_3;zeros(6,1);init_4;zeros(6,1);]  MaximumPoints=1e4  ZeroDelay=on
  ref : Outport
  "signal " : Outport  Port=2
  q : Outport  Port=3
  " Rate" : Outport  Port=4
  wires:
  Constant7/1 -> MATLAB Function3/2(alpha)
  Constant/1 -> MATLAB Function3/3(A)
  Constant1/1 -> MATLAB Function3/4(i)
  MATLAB Function3/1(vi) -> ref/1
  Integrator Limited2/1 -> Scope1/1, Divide2/1, q/1  "q"
  Switch/1 -> "signal "/1, Scope6/1, MATLAB Function3/1(x)
  u/1 -> Variable Time Delay/1
  Sum2/1 -> Integrator Limited2/1  "q_dot"
  Divide2/1 -> Scope/1, Variable Time Delay/2
  C/1 -> Divide2/2, Sum2/2
  Sample and Hold/1 -> Switch/1
  Add/1 -> Sum2/1, Scope2/1
  Integrator Limited1/1 -> Sum/2  "q"
  PID Controller/1 -> Sum1/1, " Rate"/1, Scope3/1
  Sum1/1 -> Integrator Limited1/1  "q_dot"
  C1/1 -> Sum1/2
  Sum/1 -> Scope4/1, PID Controller/1
  q_des/1 -> Sum/1
  " Real Rates"/1 -> Gain/1
  Gain/1 -> Demux/1
  Demux/1 -> Add/1
  Demux/2 -> Add/2
  Demux/3 -> Add/3
  Demux/4 -> Add/4
  Demux/5 -> Add/5
  Power/1 -> Equal/2
  Saturation/1 -> Equal/1
  Random Number/1 -> Saturation/1
  Constant4/1 -> Power/2
  Equal/1 -> Scope5/1, Sample and Hold/Trigger, Switch/2
  Constant3/1 -> Power/1
  Variable Time Delay/1 -> Sample and Hold/1, Switch/3

== system Communication_rate_control/trasmission/Subsystem1 ==
  Data : Inport
  Rate : Inport  Port=2
  Constant13 : Constant
  Constant2 : Constant
  Divide : Product  Inputs=*/
  Integrator : Integrator  ExternalReset=rising
  Relational Operator : RelationalOperator  Operator=<=  OutDataTypeStr=boolean  RndMeth=Simplest  InputSameDT=off
  Sample and Hold5 : dspsigops/Sample and Hold  trig=Rising edge  initCond=0  latchinput=off
  Unit Delay : UnitDelay  SampleTime=Ts  HasFrameUpgradeWarning=on
  "Samples " : Outport
  wires:
  Data/1 -> Sample and Hold5/1
  Constant2/1 -> Integrator/1
  Rate/1 -> Divide/2
  Unit Delay/1 -> Integrator/2
  Constant13/1 -> Divide/1
  Divide/1 -> Relational Operator/1
  Relational Operator/1 -> Unit Delay/1, Sample and Hold5/Trigger
  Sample and Hold5/1 -> "Samples "/1
  Integrator/1 -> Relational Operator/2

== system Communication_rate_control/trasmission/Subsystem2 ==
  note: Subsystem13
  In : Inport
  In1 : Inport  Port=2
  Constant13 : Constant
  Constant2 : Constant
  Divide : Product  Inputs=*/
  Integrator : Integrator  ExternalReset=rising
  Relational Operator : RelationalOperator  Operator=<=  OutDataTypeStr=boolean  RndMeth=Simplest  InputSameDT=off
  Sample and Hold5 : dspsigops/Sample and Hold  trig=Rising edge  initCond=0  latchinput=off
  Scope3 : Scope
      settings: ActiveDisplayYMinimum=-3.131696080231905E+7  ActiveDisplayYMaximum=3.596063759040764E+7  DataLoggingVariableName=ScopeData9
  Unit Delay : UnitDelay  SampleTime=Ts  HasFrameUpgradeWarning=on
  " " : Outport
  wires:
  In/1 -> Sample and Hold5/1
  Constant2/1 -> Integrator/1
  In1/1 -> Divide/2
  Unit Delay/1 -> Integrator/2
  Constant13/1 -> Divide/1
  Divide/1 -> Relational Operator/1, Scope3/1
  Relational Operator/1 -> Unit Delay/1, Sample and Hold5/Trigger
  Sample and Hold5/1 -> " "/1
  Integrator/1 -> Relational Operator/2

== system Communication_rate_control/trasmission/Subsystem3 ==
  note: Subsystem13
  In : Inport
  In1 : Inport  Port=2
  Constant13 : Constant
  Constant2 : Constant
  Divide : Product  Inputs=*/
  Integrator : Integrator  ExternalReset=rising
  Relational Operator : RelationalOperator  Operator=<=  OutDataTypeStr=boolean  RndMeth=Simplest  InputSameDT=off
  Sample and Hold5 : dspsigops/Sample and Hold  trig=Rising edge  initCond=0  latchinput=off
  Scope3 : Scope
      settings: ActiveDisplayYMinimum=-3.131696080231905E+7  ActiveDisplayYMaximum=3.596063759040764E+7  DataLoggingVariableName=ScopeData9
  Unit Delay : UnitDelay  SampleTime=Ts  HasFrameUpgradeWarning=on
  " " : Outport
  wires:
  Integrator/1 -> Relational Operator/2
  Sample and Hold5/1 -> " "/1
  Relational Operator/1 -> Sample and Hold5/Trigger, Unit Delay/1
  Divide/1 -> Scope3/1, Relational Operator/1
  Constant13/1 -> Divide/1
  Unit Delay/1 -> Integrator/2
  In1/1 -> Divide/2
  Constant2/1 -> Integrator/1
  In/1 -> Sample and Hold5/1

== system Communication_rate_control/trasmission/Subsystem4 ==
  note: Subsystem13
  In : Inport
  In1 : Inport  Port=2
  Constant13 : Constant
  Constant2 : Constant
  Divide : Product  Inputs=*/
  Integrator : Integrator  ExternalReset=rising
  Relational Operator : RelationalOperator  Operator=<=  OutDataTypeStr=boolean  RndMeth=Simplest  InputSameDT=off
  Sample and Hold5 : dspsigops/Sample and Hold  trig=Rising edge  initCond=0  latchinput=off
  Scope3 : Scope
      settings: ActiveDisplayYMinimum=-3.131696080231905E+7  ActiveDisplayYMaximum=3.596063759040764E+7  DataLoggingVariableName=ScopeData9
  Unit Delay : UnitDelay  SampleTime=Ts  HasFrameUpgradeWarning=on
  " " : Outport
  wires:
  In/1 -> Sample and Hold5/1
  Constant2/1 -> Integrator/1
  In1/1 -> Divide/2
  Unit Delay/1 -> Integrator/2
  Constant13/1 -> Divide/1
  Divide/1 -> Relational Operator/1, Scope3/1
  Relational Operator/1 -> Unit Delay/1, Sample and Hold5/Trigger
  Sample and Hold5/1 -> " "/1
  Integrator/1 -> Relational Operator/2

== system Communication_rate_control/trasmission/Subsystem5 ==
  note: Subsystem13
  In : Inport
  In1 : Inport  Port=2
  Constant13 : Constant
  Constant2 : Constant
  Divide : Product  Inputs=*/
  Integrator : Integrator  ExternalReset=rising
  Relational Operator : RelationalOperator  Operator=<=  OutDataTypeStr=boolean  RndMeth=Simplest  InputSameDT=off
  Sample and Hold5 : dspsigops/Sample and Hold  trig=Rising edge  initCond=0  latchinput=off
  Scope3 : Scope
      settings: ActiveDisplayYMinimum=-3.131696080231905E+7  ActiveDisplayYMaximum=3.596063759040764E+7  DataLoggingVariableName=ScopeData9
  Unit Delay : UnitDelay  SampleTime=Ts  HasFrameUpgradeWarning=on
  " " : Outport
  wires:
  Integrator/1 -> Relational Operator/2
  Sample and Hold5/1 -> " "/1
  Relational Operator/1 -> Sample and Hold5/Trigger, Unit Delay/1
  Divide/1 -> Scope3/1, Relational Operator/1
  Constant13/1 -> Divide/1
  Unit Delay/1 -> Integrator/2
  In1/1 -> Divide/2
  Constant2/1 -> Integrator/1
  In/1 -> Sample and Hold5/1

== system Communication_rate_control/Subsystem1/Subsystem_1/Inner-loop control ==
  zb_des : Inport
  Rb : Inport  Port=2
  omega_bb : Inport  Port=3
  xb_des : Inport  Port=4
  Derivation : DiscreteTransferFcn  Numerator=[1 -1]  Denominator=[Ts 0]  InitialStates=[1 0 0;0 1 0;0 0 1]  SampleTime=Ts
  Derivation1 : DiscreteTransferFcn  Numerator=[1 -1]  Denominator=[Ts 0]  InitialStates=[0 0 0]  SampleTime=Ts
  Inner-loop control : MATLAB Function  TreatAsAtomicUnit=on
  Unit Delay1 : UnitDelay  InitialCondition=eye(3)  SampleTime=Ts
  Unit Delay3 : UnitDelay  InitialCondition=[0 0 0]  SampleTime=Ts
  tau : Outport
  err_R : Outport  Port=2
  err_W : Outport  Port=3
  wires:
  Inner-loop control/2(omega_bb_des) -> Derivation1/1
  Inner-loop control/1(Rb_des) -> Derivation/1
  omega_bb/1 -> Inner-loop control/4(omega_bb)
  zb_des/1 -> Inner-loop control/1(zb_des)
  Derivation/1 -> Unit Delay1/1
  Unit Delay3/1 -> Inner-loop control/5(dot_omega_bb_des)
  Inner-loop control/5(err_W) -> err_W/1
  Derivation1/1 -> Unit Delay3/1
  Unit Delay1/1 -> Inner-loop control/3(dot_Rb_des)
  Inner-loop control/3(tau) -> tau/1
  Rb/1 -> Inner-loop control/2(Rb)
  Inner-loop control/4(err_R) -> err_R/1
  xb_des/1 -> Inner-loop control/6(xb_des)

== system Communication_rate_control/Subsystem1/Subsystem_1/Planner ==
  References : Inport
  Constant : Constant  Value=0
  Demux : Demux  Outputs=10
  Mux{1..4} (4 alike) : Mux  Inputs=3
  Trigonometric Function : Trigonometry
  Trigonometric Function1 : Trigonometry  Operator=cos
  position_des : Outport
  linear_velocity_des : Outport  Port=2
  linear_acceleration_des : Outport  Port=3
  xb_des : Outport  Port=4
  wires:
  References/1 -> Demux/1
  Demux/10 -> Trigonometric Function1/1, Trigonometric Function/1
  Demux/9 -> Mux1/3
  Demux/8 -> Mux1/2
  Demux/7 -> Mux1/1
  Demux/6 -> Mux3/3
  Demux/5 -> Mux3/2
  Demux/4 -> Mux3/1
  Demux/3 -> Mux2/3
  Demux/2 -> Mux2/2
  Demux/1 -> Mux2/1
  Constant/1 -> Mux4/3
  Trigonometric Function1/1 -> Mux4/1
  Trigonometric Function/1 -> Mux4/2
  Mux4/1 -> xb_des/1
  Mux2/1 -> position_des/1
  Mux3/1 -> linear_velocity_des/1
  Mux1/1 -> linear_acceleration_des/1

== system Communication_rate_control/Subsystem1/Subsystem_1/Quadrotor dynamics ==
  uT : Inport
  tau_b : Inport  Port=2
  Integrator : Integrator  InitialCondition=init_0
  Integrator1 : Integrator  InitialCondition=lin_vel_0
  Integrator2 : Integrator  InitialCondition=[1 0 0; 0 1 0;0 0 1]
  Integrator3 : Integrator  InitialCondition=w_bb_0
  MATLAB Function1 : MATLAB Function  TreatAsAtomicUnit=on
  UAV dynamics : MATLAB Function  TreatAsAtomicUnit=on
  Position : Outport
  Linear_velocity : Outport  Port=2
  Rb : Outport  Port=3
  dot_Rb : Outport  Port=4
  omega_bb : Outport  Port=5
  dot_omega_bb : Outport  Port=6
  lin_acc : Outport  Port=7
  wires:
  Integrator2/1 -> MATLAB Function1/1(Rb_temp)
  MATLAB Function1/1(Rb) -> UAV dynamics/3(Rb), Rb/1
  UAV dynamics/2(dot_Rb) -> dot_Rb/1, Integrator2/1
  Integrator3/1 -> omega_bb/1, UAV dynamics/4(omega_bb)
  Integrator1/1 -> Integrator/1, Linear_velocity/1
  uT/1 -> UAV dynamics/1(uT)
  UAV dynamics/1(lin_acc) -> Integrator1/1, lin_acc/1
  UAV dynamics/3(ang_acc) -> Integrator3/1, dot_omega_bb/1
  Integrator/1 -> Position/1
  tau_b/1 -> UAV dynamics/2(tau_b)
